simulink model "Y3Tiltrotor_sim3_INDI"  (R2025a)
settings: Solver=ode4  StartTime=0.0  StopTime=70  FixedStep=uavParam.sampleTime  RelTol=1e-3
PreLoadFcn:
  | filepath  = fileparts(get_param(bdroot, 'FileName'))
  | cd(filepath);
InitFcn:
  | Init_sim_INDI;
values from neighbouring files (symbols this model uses):
  control = struct    [Init_sim_INDI.m]
  env = struct    [InitData.m]
  flightState = struct    [Init_sim_INDI.m]
  FWSpeed0 = 15    [Init_sim_INDI.m]
  k_lpf_p = 50    [Init_sim_INDI.m]
  k_lpf_q = 80    [Init_sim_INDI.m]
  k_lpf_r = 5    [Init_sim_INDI.m]
  k_lpf_u = 10    [Init_sim_INDI.m]
  k_lpf_v = 1    [Init_sim_INDI.m]
  k_lpf_w = 50    [Init_sim_INDI.m]
  k_p = 5    [Init_sim_INDI.m]
  k_q = 20    [Init_sim_INDI.m]
  k_r = 1.5    [Init_sim_INDI.m]
  k_u = 0.5    [Init_sim_INDI.m]
  k_v = 0.5    [Init_sim_INDI.m]
  k_w = 2    [Init_sim_INDI.m]
  uavParam = struct    [InitData.m]
undefined symbols (not defined in the file or in its folder): ControlSampleTime, F, Light, MIL, Newton, Raphson
libraries: slpidlib x28, SignalEditorBlockLib x12, simulink x6, aerolibtransform2 x3, sharedtransform x3, robotcorelib x3, matrix_library x3, aerolibasang x2, aerolibutil x2, aerolibwind2 x2, shared6dof x1, aerolibatmos2 x1
(part 1 of 7)
settings Model: Creator=YuXinchen  LastModifiedBy=11696
settings SolverCC: AlgebraicLoopSolver=TrustRegion
settings DataIOCC: ReturnWorkspaceOutputs=off
settings DebuggingCC: UnconnectedInputMsg=warning  UnconnectedOutputMsg=warning  UnconnectedLineMsg=warning  UnderSpecifiedDimensionMsg=warning
settings ModelReferenceCC: EnableRefExpFcnMdlSchedulingChecks=on
settings RTWCC: GPUComputeCapability=3.5  DLArmComputeVersion=19.05

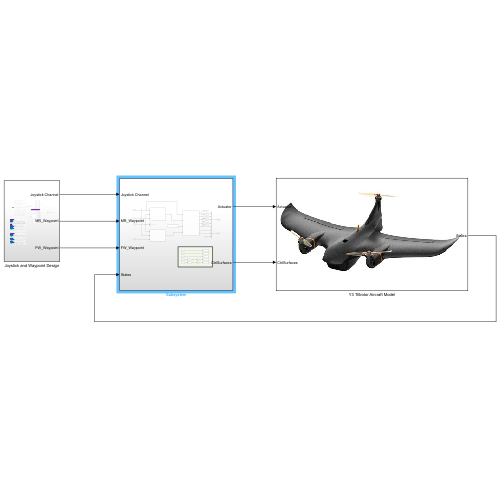
[thumbnail: Simulink's stored preview of the top-level diagram]
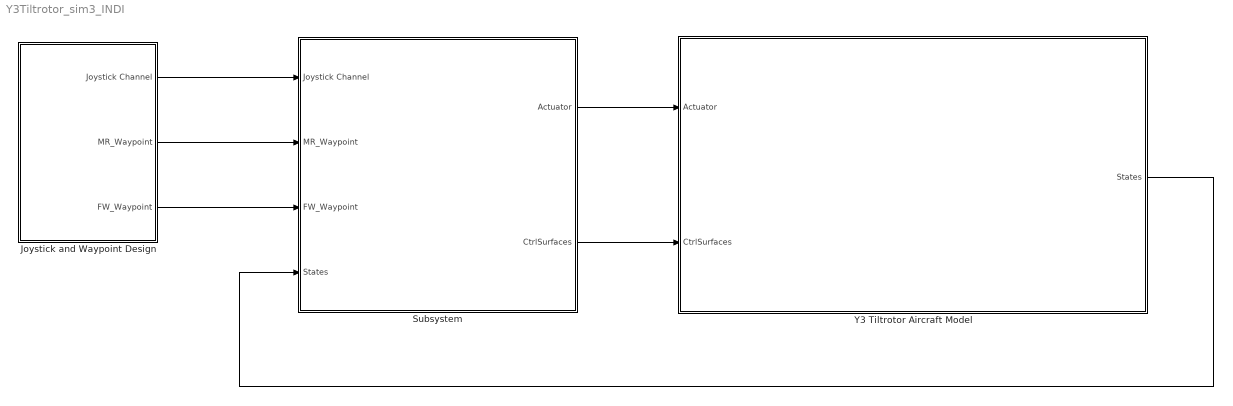
== system Y3Tiltrotor_sim3_INDI ==
  Joystick and Waypoint Design : Subsystem
  Subsystem : Subsystem
  Y3 Tiltrotor Aircraft Model : Subsystem
      mask Display: image('Y3Tiltrotor.jpg');
  wires:
  Subsystem/1(Actuator) -> Y3 Tiltrotor Aircraft Model/1(Actuator)
  Subsystem/2(CtrlSurfaces) -> Y3 Tiltrotor Aircraft Model/2(CtrlSurfaces)
  Y3 Tiltrotor Aircraft Model/1(States) -> Subsystem/4(States)
  Joystick and Waypoint Design/1(Joystick Channel) -> Subsystem/1(Joystick Channel)
  Joystick and Waypoint Design/2(MR_Waypoint) -> Subsystem/2(MR_Waypoint)
  Joystick and Waypoint Design/3(FW_Waypoint) -> Subsystem/3(FW_Waypoint)

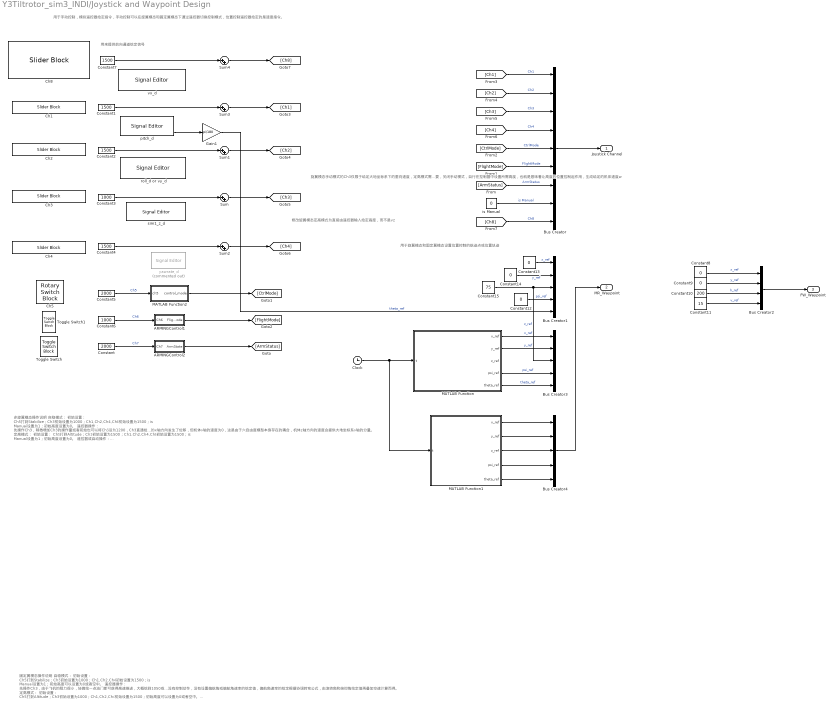
== system Y3Tiltrotor_sim3_INDI/Joystick and Waypoint Design ==
  note: 旋翼模态手动模式的Ch3仅限于给定大地坐标系下的垂向速度，定高模式需要，关闭手动模式，自行在控制器中设置所需高度，也就是意味着让高度的位置控制起作用，生成给定的机体速度w
  note: 用来提供前向通道给定信号
  note: 用于手动控制，模拟遥控器给定指令，手动控制可以在旋翼模态和固定翼模态下通过遥控器切换控制模式，位置控制遥控器给定的是速度指令。
  note: 用于旋翼模态和固定翼模态设置位置控制的航迹点或位置轨迹
  note: 固定翼模态操作说明
      |
      | 自稳模式：
      | 初始设置： Ch5打到Stabilize；Ch3初始设置为1000；Ch1,Ch2,Ch4初始设置为1500；is Manual设置为1；初始高度可以设置为0或者空中。
      | 遥控器操作： 先操作Ch3，由于飞机的阻力很小，轻微给一点油门即可获得高速推进，大概给到1050或1100即可；Ch1控制俯仰运动，在有油门的情况下进行操纵，增大Ch1即增大给定俯仰角，反之减小，抬头为正，低头为负；Ch2控制滚转运动，在有油门的情况下进行操纵，增大Ch2即增大给定滚转角，反之减小，向右滚转为正，向左滚转为负；Ch4没有控制动作，没有设置偏航角或偏航角速率的给定值，偏航角速率的给定根据协调转弯公式，由滚转角和俯仰角给定值再叠加空速计算而得。
      | 定高模式：
      | 初始设置： Ch5打到Altitude；Ch3初始设置为1000；Ch1,Ch2,Ch4初始设置为1500；初始高度可以设置为0或者空中。
      | 遥控器或自动操作： 此模式下无论是遥控器还是自动飞行，Ch3的操作和自稳模式一致；Ch2和Ch4的操作和自稳模式一致。当is Manual设置为1时（手动），Ch1控制飞机的垂向速度，增大Ch1即增大给定垂向速度，反之减小；当is Manual设置为0时（自动），Ch1不起作用，由FW_Waypoint给定飞机的飞行高度h_ref，高度控制器中的高度位置控制起作用。
      | 定速模式 ：
      | 初始设置： Ch5打到Position；Ch3初始设置可以为1000；Ch1,Ch2,Ch4初始设置为1500；初始高度可以设置为0或者空中。
      | 遥控器或自动操作： 此模式下无论是遥控器还是自动飞行，Ch2和Ch4的操作和自稳模式一致。当is Manual设置为1时（手动），Ch3控制飞机的空速，定速模式遥控器给定空速变化范围设置为15-25m/s；Ch1控制飞机的垂向速度，增大Ch1即增大给定垂向速度，反之减小。当is Manual设置为0时（自动），Ch1和Ch3都不起作用，对应于定速模式的给定变成了由FW_Waypoint给定飞机的飞行高度h_ref和飞行速度v_ref，在自动模式下，也可以调整CoupledControl的值来设置是否开启总能量控制。
  note: 多旋翼模态操作说明
      |
      | 自稳模式：
      | 初始设置： Ch5打到Stabilize；Ch3初始设置为1000；Ch1,Ch2,Ch4,Ch8初始设置为1500；is Manual设置为1；初始高度设置为0。
      | 遥控器操作： 先操作Ch3，稍微增加Ch3的操作量或者初始也可以将Ch3设为1200，Ch3直通给到油门量，飞行器将获得持续的推力，当达到想要的高度后可以适当降低油门量使其能大致平衡重力，也可以保持垂向飞行的状态操作其他通道。Ch1控制俯仰通道，给定俯仰角；Ch2控制滚转通道，给定滚转角；Ch4控制偏航通道，给定偏航角速率，Ch8控制前向通道，给定机体坐标系前向速度。由于所设计的控制逻辑是通过前两个旋翼的油门和倾转角来控制前向通道，与俯仰通道解耦，所以在自稳模式的前向通道控制过程中，俯仰角可以始终为0，可以自行设定；在俯仰通道的控制过程中，前向速度也可以设定为0，但通常会发现无人机的x轴方向发生了位移，但机体x轴的速度为0，这是由于六自由度模型本身存在的耦合，机体z轴方向的速度会提供大地坐标系x轴的分量。
      | 定高模式：
      | 初始设置： Ch5打到Altitude；Ch3初始设置为1500；Ch1,Ch2,Ch4,Ch8初始设置为1500；is Manual设置为1；初始高度设置为0。
      | 遥控器或自动操作： 此模式下只有Ch3和自稳模式不一样，其他通道基本保持一致。Ch3控制垂向速度，给定为大地坐标系下z轴的速度。其他通道做动作时，通常将Ch3置为1500，即将无人机保持定高飞行，高度不变的情况下做其他动作。
      | 定点模式 ：
      | 初始设置： Ch5打到Position；Ch3初始设置可以为1500；Ch1,Ch2,Ch4 ,Ch8 初始设置为1500；初始高度可以设置为0。
      | 遥控器或自动操作： 此模式下无论是遥控器还是自动飞行，Ch1和Ch4,Ch8的操作和自稳模式一致。当is Manual设置为1时（手动），Ch3控制垂向速度，和定高模式保持一致；Ch2控制横侧向通道，给定为飞机机体坐标系y轴的速度（横向速度）。当is Manual设置为0时（自动），Ch1, Ch2, Ch3 ,Ch4 ,Ch8都不起作用，对应于定速模式的给定变成了由FW_Waypoint给定飞机的x_ref,y_ref,z_ref,psi_ref的给定。
  note: 修改旋翼模态定高模式为直接由遥控器输入给定高度，而不是vz
  ARMINGControl1 : Subsystem
  ARMINGControl2 : Subsystem
  Bus Creator : BusCreator  Inputs=9
  Bus Creator1 : BusCreator  Inputs=5
  Bus Creator2 : BusCreator  Inputs=4
  Bus Creator3 : BusCreator  Inputs=5
  Bus Creator4 : BusCreator  Inputs=5
  Ch{1..4,8} (5 alike) : SliderBlock  ScaleMin=1000  ScaleMax=2000  TickInterval=200
  Ch5 : RotarySwitchBlock
  Clock : Clock
  Constant : Constant  Value=2000
  Constant{1..2,4,7} (4 alike) : Constant  Value=1500
  Constant10 : Constant  Value=200
  Constant11 : Constant  Value=15
  Constant{8..9,12..14} (5 alike) : Constant  Value=0
  Constant15 : Constant  Value=75
  Constant3 : Constant  Value=1000
  Constant5 : Constant  Value=2000
  Constant6 : Constant  Value=1000
  Gain1 : Gain  Gain=pi/180
  MATLAB Function : MATLAB Function  TreatAsAtomicUnit=on
  MATLAB Function1 : MATLAB Function  TreatAsAtomicUnit=on
  MATLAB Function2 : MATLAB Function  TreatAsAtomicUnit=on
  Sum{,1..4} (5 alike) : Sum  Inputs=|++
  Toggle Switch : ToggleSwitchBlock
  Toggle Switch1 : ToggleSwitchBlock
  is Manual : Constant  Value=0
  pitch_d : SignalEditorBlockLib/Signal Editor  FileName=pitch_d.mat  ActiveScenario=Test  ActiveSignal=俯仰角测试-遥控器  IsBus=off  OutputBusObjectStr=Bus: BusObject  SampleTime=0  ZeroCross=off  OutputAfterFinalValue=Setting to zero  Unit=inherit  PreserveSignalName=on  ApplySigPropsToAllScenarios=on  ApplySigPropsToAllSignals=on  SignalPropertySource=Dialog parameters
  roll_d or vy_d : SignalEditorBlockLib/Signal Editor  FileName=roll_d.mat  ActiveScenario=Test  ActiveSignal=定高-滚转角测试-遥控器  IsBus=off  OutputBusObjectStr=Bus: BusObject  SampleTime=0  ZeroCross=off  OutputAfterFinalValue=Setting to zero  Unit=inherit  PreserveSignalName=on  ApplySigPropsToAllScenarios=on  ApplySigPropsToAllSignals=on  SignalPropertySource=Dialog parameters
  sim1_z_d : SignalEditorBlockLib/Signal Editor  FileName=vz_d.mat  ActiveScenario=Test  ActiveSignal=直接给定高度-遥控器  IsBus=off  OutputBusObjectStr=Bus: BusObject  SampleTime=0  ZeroCross=off  OutputAfterFinalValue=Setting to zero  Unit=inherit  PreserveSignalName=on  ApplySigPropsToAllScenarios=on  ApplySigPropsToAllSignals=on  SignalPropertySource=Dialog parameters
  vx_d : SignalEditorBlockLib/Signal Editor  FileName=vx_d.mat  ActiveScenario=Test  ActiveSignal=定点-前向速度测试-遥控器  IsBus=off  OutputBusObjectStr=Bus: BusObject  SampleTime=0  ZeroCross=off  OutputAfterFinalValue=Setting to zero  Unit=inherit  PreserveSignalName=on  ApplySigPropsToAllScenarios=on  ApplySigPropsToAllSignals=off  SignalPropertySource=Dialog parameters
  yawrate_d : SignalEditorBlockLib/Signal Editor  Commented=on  FileName=untitled.mat  ActiveScenario=Scenario  ActiveSignal=Signal 1  IsBus=off  OutputBusObjectStr=Bus: BusObject  SampleTime=0  ZeroCross=off  OutputAfterFinalValue=Setting to zero  Unit=inherit  PreserveSignalName=on  ApplySigPropsToAllScenarios=on  ApplySigPropsToAllSignals=off  SignalPropertySource=Dialog parameters
  Joystick Channel : Outport
  MR_Waypoint : Outport  Port=2
  FW_Waypoint : Outport  Port=3
  wires:
  Constant5/1 -> MATLAB Function2/1(ch5)  "Ch5"
  Constant/1 -> ARMINGControl2/1(Ch7)  "Ch7"
  Constant6/1 -> ARMINGControl1/1(Ch6)  "Ch6"
  ARMINGControl2/1(ArmState) -> [ArmStatus]
  MATLAB Function2/1(control_mode) -> [CtrlMode]
  ARMINGControl1/1(FlightMode) -> [FlightMode]
  Bus Creator/1 -> Joystick Channel/1
  [CtrlMode] -> Bus Creator/5  "CtrlMode"
  [FlightMode] -> Bus Creator/6  "FlightMode"
  [ArmStatus] -> Bus Creator/7  "ArmStatus"
  [Ch1] -> Bus Creator/1  "Ch1"
  [Ch2] -> Bus Creator/2  "Ch2"
  [Ch3] -> Bus Creator/3  "Ch3"
  [Ch4] -> Bus Creator/4  "Ch4"
  is Manual/1 -> Bus Creator/8  "is Manual"
  Constant3/1 -> Sum/1
  Constant2/1 -> Sum1/1
  Constant4/1 -> Sum2/1
  Sum1/1 -> [Ch2]
  Sum/1 -> [Ch3]
  Sum2/1 -> [Ch4]
  Sum3/1 -> [Ch1]
  Constant1/1 -> Sum3/1
  [Ch8] -> Bus Creator/9  "Ch8"
  Sum4/1 -> [Ch8]
  Constant7/1 -> Sum4/1
  Constant14/1 -> Bus Creator1/2  "y_ref"
  Constant13/1 -> Bus Creator1/1  "x_ref"
  Clock/1 -> MATLAB Function1/1(t), MATLAB Function/1(t)
  Constant12/1 -> Bus Creator1/4  "psi_ref"
  Constant11/1 -> Bus Creator2/4  "v_ref"
  Constant8/1 -> Bus Creator2/1  "x_ref"
  Constant10/1 -> Bus Creator2/3  "h_ref"
  Bus Creator2/1 -> FW_Waypoint/1
  Constant9/1 -> Bus Creator2/2  "y_ref"
  Constant15/1 -> Bus Creator1/3, Bus Creator3/3  "z_ref"
  pitch_d/3 -> Gain1/1
  Gain1/1 -> Bus Creator1/5  "theta_ref"
  MATLAB Function/1(x_ref) -> Bus Creator3/1  "x_ref"
  MATLAB Function/2(y_ref) -> Bus Creator3/2  "y_ref"
  MATLAB Function/4(psi_ref) -> Bus Creator3/4  "psi_ref"
  MATLAB Function/5(theta_ref) -> Bus Creator3/5  "theta_ref"
  MATLAB Function1/3(z_ref) -> Bus Creator4/3
  MATLAB Function1/1(x_ref) -> Bus Creator4/1
  MATLAB Function1/2(y_ref) -> Bus Creator4/2
  MATLAB Function1/4(psi_ref) -> Bus Creator4/4
  MATLAB Function1/5(theta_ref) -> Bus Creator4/5
  Bus Creator4/1 -> MR_Waypoint/1

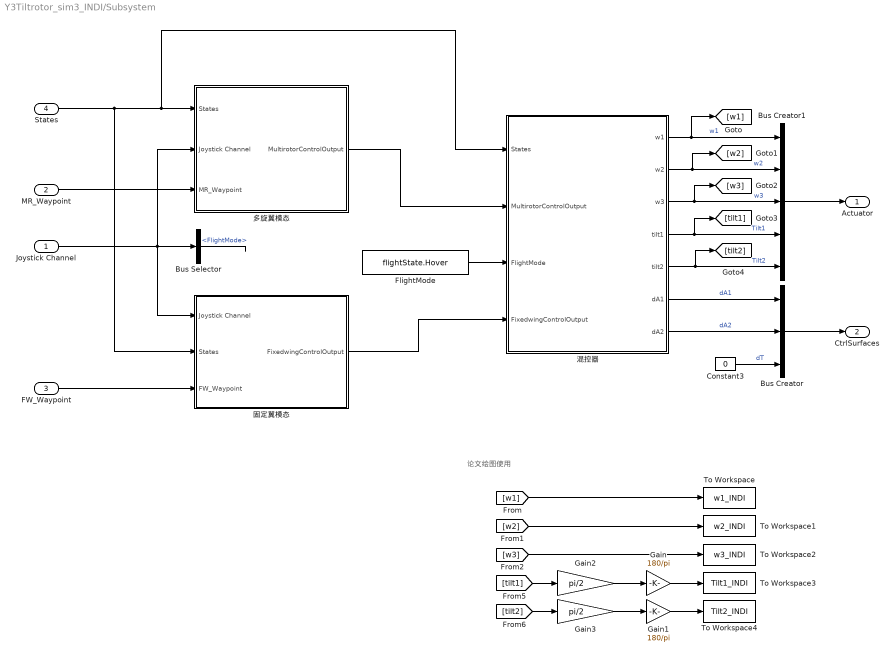
== system Y3Tiltrotor_sim3_INDI/Subsystem ==
  note: 论文绘图使用
  Joystick Channel : Inport
  MR_Waypoint : Inport  Port=2
  FW_Waypoint : Inport  Port=3
  States : Inport  Port=4
  Bus Creator : BusCreator  Inputs=3
  Bus Creator1 : BusCreator  Inputs=5
  Bus Selector : BusSelector  OutputSignals=FlightMode
  Constant3 : Constant  Value=0
  FlightMode : Constant  Value=flightState.Hover
  Gain : Gain  Gain=180/pi
  Gain1 : Gain  Gain=180/pi
  Gain2 : Gain  Gain=pi/2
  Gain3 : Gain  Gain=pi/2
  To Workspace : ToWorkspace  VariableName=w1_INDI  SampleTime=-1
      settings: Save2DSignal=2-D array (concatenate along first dimension)
  To Workspace1 : ToWorkspace  VariableName=w2_INDI  SampleTime=-1
      settings: Save2DSignal=2-D array (concatenate along first dimension)
  To Workspace2 : ToWorkspace  VariableName=w3_INDI  SampleTime=-1
      settings: Save2DSignal=2-D array (concatenate along first dimension)
  To Workspace3 : ToWorkspace  VariableName=Tilt1_INDI  SampleTime=-1
      settings: Save2DSignal=2-D array (concatenate along first dimension)
  To Workspace4 : ToWorkspace  VariableName=Tilt2_INDI  SampleTime=-1
      settings: Save2DSignal=2-D array (concatenate along first dimension)
  固定翼模态 : Subsystem
  多旋翼模态 : Subsystem
  混控器 : Subsystem
  Actuator : Outport
  CtrlSurfaces : Outport  Port=2
  wires:
  Constant3/1 -> Bus Creator/3  "dT"
  混控器/5(tilt2) -> [tilt2], Bus Creator1/5  "Tilt2"
  混控器/4(tilt1) -> [tilt1], Bus Creator1/4  "Tilt1"
  Bus Creator/1 -> CtrlSurfaces/1
  Bus Creator1/1 -> Actuator/1
  States/1 -> 混控器/1(States), 多旋翼模态/1(States), 固定翼模态/2(States)
  混控器/1(w1) -> [w1], Bus Creator1/1  "w1"
  混控器/2(w2) -> [w2], Bus Creator1/2  "w2"
  混控器/3(w3) -> [w3], Bus Creator1/3  "w3"
  混控器/7(dA2) -> Bus Creator/2  "dA2"
  混控器/6(dA1) -> Bus Creator/1  "dA1"
  FlightMode/1 -> 混控器/3(FlightMode)
  Joystick Channel/1 -> Bus Selector/1, 多旋翼模态/2(Joystick Channel), 固定翼模态/1(Joystick Channel)
  Bus Selector/1 -> ?  "<FlightMode>"
  MR_Waypoint/1 -> 多旋翼模态/3(MR_Waypoint)
  FW_Waypoint/1 -> 固定翼模态/3(FW_Waypoint)
  多旋翼模态/1(MultirotorControlOutput) -> 混控器/2("MultirotorControlOutput ")
  固定翼模态/1(FixedwingControlOutput) -> 混控器/4("FixedwingControlOutput ")
  Gain3/1 -> Gain1/1
  Gain2/1 -> Gain/1
  Gain1/1 -> To Workspace4/1
  [w1] -> To Workspace/1
  [w2] -> To Workspace1/1
  [w3] -> To Workspace2/1
  Gain/1 -> To Workspace3/1
  [tilt2] -> Gain3/1
  [tilt1] -> Gain2/1

== system Y3Tiltrotor_sim3_INDI/Y3 Tiltrotor Aircraft Model ==
  Actuator : Inport
  CtrlSurfaces : Inport  Port=2
  6DOF (Euler Angles) : shared6dof/6DOF (Euler Angles)  units=Metric (MKS)  mtype=Fixed  rep=Euler Angles  xme_0=ModelInit_PosE  Vm_0=ModelInit_VelB  eul_0=ModelInit_AngEuler  pm_0=ModelInit_RateB  mass_0=uavParam.geom.mass  mass_e=0.5  mass_f=2.0  inertia=eye(3).*[uavParam.inertia.Ixx; uavParam.inertia.Iyy; uavParam.inertia.Izz]  inertia_e=eye(3)  inertia_f=2*eye(3)  k_quat=1.0  vre_flag=on  abi_flag=off  aMode=aMode  xme_statename=''  Vm_statename=''  eul_statename=''  quat_statename=''  pm_statename=''  mass_statename=''
  Rate Transition : RateTransition
  Rate Transition1 : RateTransition
  States Bus : Subsystem
  Subsystem : Subsystem
  States : Outport
  wires:
  6DOF (Euler Angles)/1 -> States Bus/1(Ve)  "Ve"
  States Bus/1(States) -> Subsystem/3(States), States/1
  6DOF (Euler Angles)/8 -> States Bus/8(Abb)  "Abb"
  6DOF (Euler Angles)/7 -> States Bus/7(dw/dt)  "dw/dt"
  6DOF (Euler Angles)/6 -> States Bus/6(pqr)  "pqr"
  6DOF (Euler Angles)/5 -> States Bus/5(Vb)  "Vb"
  6DOF (Euler Angles)/4 -> States Bus/4(DCMbe)  "DCM"
  6DOF (Euler Angles)/3 -> States Bus/3(Euler)  "Euler"
  6DOF (Euler Angles)/2 -> States Bus/2(Xe)  "Xe"
  CtrlSurfaces/1 -> Rate Transition1/1
  Actuator/1 -> Rate Transition/1
  Subsystem/1(Fb) -> 6DOF (Euler Angles)/1  "F_b"
  Subsystem/2(Mb) -> 6DOF (Euler Angles)/2  "M_b"
  Subsystem/3(RotorParams) -> States Bus/9(RotorParams)
  Subsystem/4(Airspeed) -> States Bus/10(Airspeed)
  Rate Transition1/1 -> Subsystem/2(CtrlSurfaces)
  Rate Transition/1 -> Subsystem/1(Actuator)

== system Y3Tiltrotor_sim3_INDI/Joystick and Waypoint Design/ARMINGControl1 ==
  Ch6 : Inport
  Compare To Constant3 : simulink/Logic and Bit Operations/Compare To Constant  relop=>=  const=uint16(1400)  OutDataTypeStr=boolean
  FlightMode : Outport  VectorParamsAs1DForOutWhenUnconnected=off
  wires:
  Ch6/1 -> Compare To Constant3/1
  Compare To Constant3/1 -> FlightMode/1

== system Y3Tiltrotor_sim3_INDI/Joystick and Waypoint Design/ARMINGControl2 ==
  Ch7 : Inport
  Compare To Constant3 : simulink/Logic and Bit Operations/Compare To Constant  relop=>=  const=uint16(1400)  OutDataTypeStr=boolean
  ArmState : Outport  VectorParamsAs1DForOutWhenUnconnected=off
  wires:
  Compare To Constant3/1 -> ArmState/1
  Ch7/1 -> Compare To Constant3/1

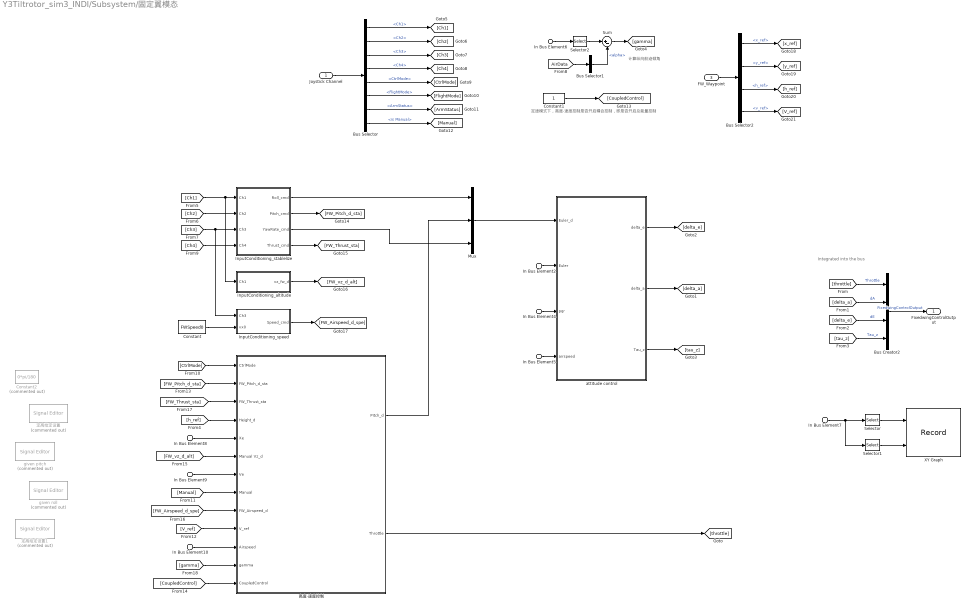
== system Y3Tiltrotor_sim3_INDI/Subsystem/固定翼模态 ==
  note: 计算纵向航迹倾角
  note: Integrated into the bus
  note: 定速模式下，高度-速度控制是否开启耦合控制，即是否开启总能量控制
  Joystick Channel : Inport
  In Bus Element5 : Inport  Port=2  PortName=States  Element=Airspeed
  In Bus Element10 : Inport  Port=2  PortName=States  Element=Airspeed
  In Bus Element7 : Inport  Port=2  PortName=States  Element=Xe
  In Bus Element8 : Inport  Port=2  PortName=States  Element=Xe
  In Bus Element2 : Inport  Port=2  PortName=States  Element=Euler
  In Bus Element6 : Inport  Port=2  PortName=States  Element=Euler
  In Bus Element9 : Inport  Port=2  PortName=States  Element=Ve
  In Bus Element4 : Inport  Port=2  PortName=States  Element=pqr
  FW_Waypoint : Inport  Port=3
  Bus Creator2 : BusCreator  Inputs=4
  Bus Selector : BusSelector  OutputSignals=Ch1,Ch2,Ch3,Ch4,CtrlMode,FlightMode,ArmStatus,is Manual
  Bus Selector1 : BusSelector  OutputSignals=alpha
  Bus Selector2 : BusSelector  OutputSignals=x_ref,y_ref,h_ref,v_ref
  Constant : Constant  Value=FWSpeed0
  Constant1 : Constant
  Constant2 : Constant  Commented=on  Value=0*pi/180
  InputConditioning_altitude : Subsystem
  InputConditioning_speed : Subsystem
  InputConditioning_stablelize : Subsystem
  Mux : Mux  Inputs=3
  Selector : Selector  InputPortWidth=3  IndexOptions=Index vector (dialog)  Indices=1  OutputSizes=1
  Selector1 : Selector  InputPortWidth=3  IndexOptions=Index vector (dialog)  Indices=2  OutputSizes=1
  Selector2 : Selector  InputPortWidth=3  IndexOptions=Index vector (dialog)  Indices=2  OutputSizes=1
  Sum : Sum  Inputs=|+-
  XY Graph : Record  NumPorts=2.0  FileSettingsInternal="{\"entries\":[{\"content\":{\"excelSettings\":{\"content\":{},\"type\":\"Streamout.ExcelSettings\"},\"parquetSettings\":{\"content\":{},\"type\":\"Streamout.ParquetSettings\"}},\"type\":\"Streamout.FileSettingStorage\",\"uuid\":\"\"}],\"packageUris\":[\"http:\\/\\/schema.mathworks.com\\/mf0\\/streamout_blocks\\/R2020a\"],\"version\":\"1.0\"}"  FrameSettings=[0, 0]  Layout=OverlayBottom  SignalsInternal="{\"entries\":[{\"content\":{\"signals\":[{\"content\":{\"blockPath\":[],\"dimensions\":[1],\"domain\":\"\",\"lineColor\":\"#edb120\",\"lineWidth\":2,\"port\":1,\"sid\":[\"\"],\"signalID\":1,\"signalName\":\"Selector\"},\"type\":\"RecordBlkView.Signal\",\"uuid\":\"\"},{\"content\":{\"blockPath\":[],\"dimensions\":[1],\"domain\":\"\",\"lineColor\":\"#7e2f8e\",\"lineWidth\":2,\"port\":2,\"sid\":[\"\"],\"signalID\":2,\"signalName\":\"Selector1\"},\"type\":\"RecordBlkView.Signal\",\"uuid\":\"\"}]},\"type\":\"RecordBlkView.InputSignals\",\"uuid\":\"\"}],\"packageUris\":[\"http:\\/\\/schema.mathworks.com\\/mf0\\/streamout_blocks\\/R2020a\"],\"version\":\"1.0\"}"  VisualizationBindings="{\"xyplotplugin\":{\"info\":[{\"series\":[],\"subplotID\":1}]}}"  CompatibilityTag=XY
  attitude control : Subsystem
  given pitch : SignalEditorBlockLib/Signal Editor  Commented=on  FileName=given pitch.mat  ActiveScenario=Scenario  ActiveSignal=Signal 1  IsBus=off  OutputBusObjectStr=Bus: BusObject  SampleTime=0  Interpolate=off  ZeroCross=off  OutputAfterFinalValue=Setting to zero  Unit=inherit  PreserveSignalName=on  ApplySigPropsToAllScenarios=on  ApplySigPropsToAllSignals=off  SignalPropertySource=Dialog parameters
  given roll : SignalEditorBlockLib/Signal Editor  Commented=on  FileName=given roll.mat  ActiveScenario=Scenario  ActiveSignal=Signal 1  IsBus=off  OutputBusObjectStr=Bus: BusObject  SampleTime=-1  ZeroCross=off  OutputAfterFinalValue=Setting to zero  Unit=inherit  PreserveSignalName=on  ApplySigPropsToAllScenarios=on  ApplySigPropsToAllSignals=off  SignalPropertySource=Dialog parameters
  定高给定设置 : SignalEditorBlockLib/Signal Editor  Commented=on  FileName=E:\1-实验室相关\1-科研\10-倾转旋翼无人机\SmallTiltrotorUAV\v2.0\given Fixed Height.mat  ActiveScenario=Scenario  ActiveSignal=Signal 1  IsBus=off  OutputBusObjectStr=Bus: BusObject  SampleTime=0  ZeroCross=off  OutputAfterFinalValue=Setting to zero  Unit=inherit  PreserveSignalName=on  ApplySigPropsToAllScenarios=on  ApplySigPropsToAllSignals=off  SignalPropertySource=Dialog parameters
  定高给定设置1 : SignalEditorBlockLib/Signal Editor  Commented=on  FileName=E:\1-实验室相关\1-科研\10-倾转旋翼无人机\SmallTiltrotorUAV\v2.0\given Fixed Height.mat  ActiveScenario=Scenario  ActiveSignal=Signal 1  IsBus=off  OutputBusObjectStr=Bus: BusObject  SampleTime=0  ZeroCross=off  OutputAfterFinalValue=Setting to zero  Unit=inherit  PreserveSignalName=on  ApplySigPropsToAllScenarios=on  ApplySigPropsToAllSignals=off  SignalPropertySource=Dialog parameters
  高度-速度控制 : Subsystem
  FixedwingControlOutput : Outport
  wires:
  Mux/1 -> attitude control/1(Euler_d)
  In Bus Element2/1 -> attitude control/2(Euler)
  In Bus Element4/1 -> attitude control/3(pqr)
  attitude control/1(delta_e) -> [delta_e]
  InputConditioning_stablelize/3(YawRate_cmd) -> Mux/3
  attitude control/2(delta_a) -> [delta_a]
  attitude control/3(Tau_z) -> [tau_z]
  In Bus Element5/1 -> attitude control/4(airspeed)
  [tau_z] -> Bus Creator2/4  "Tau_z"
  [delta_e] -> Bus Creator2/3  "dE"
  [throttle] -> Bus Creator2/1  "Throttle"
  [delta_a] -> Bus Creator2/2  "dA"
  Bus Creator2/1 -> FixedwingControlOutput/1  "FixedwingControlOutput"
  Joystick Channel/1 -> Bus Selector/1
  In Bus Element6/1 -> Selector2/1
  Selector2/1 -> Sum/1
  Sum/1 -> [gamma]
  [AirData] -> Bus Selector1/1
  Bus Selector1/1 -> Sum/2  "<alpha>"
  Selector/1 -> XY Graph/1
  Selector1/1 -> XY Graph/2
  In Bus Element7/1 -> Selector1/1, Selector/1
  Bus Selector/8 -> [Manual]  "<is Manual>"
  Bus Selector/7 -> [ArmStatus]  "<ArmStatus>"
  Bus Selector/6 -> [FlightMode]  "<FlightMode>"
  Bus Selector/5 -> [CtrlMode]  "<CtrlMode>"
  Bus Selector/4 -> [Ch4]  "<Ch4>"
  Bus Selector/3 -> [Ch3]  "<Ch3>"
  Bus Selector/1 -> [Ch1]  "<Ch1>"
  Bus Selector/2 -> [Ch2]  "<Ch2>"
  Constant1/1 -> [CoupledControl]
  [Ch1] -> InputConditioning_altitude/1(Ch1), InputConditioning_stablelize/1(Ch1)
  [Ch2] -> InputConditioning_stablelize/2(Ch2)
  [Ch3] -> InputConditioning_speed/1(Ch3), InputConditioning_stablelize/3(Ch3)
  [Ch4] -> InputConditioning_stablelize/4(Ch4)
  InputConditioning_stablelize/4(Thrust_cmd) -> [FW_Thrust_sta]
  InputConditioning_stablelize/2(Pitch_cmd) -> [FW_Pitch_d_sta]
  InputConditioning_altitude/1(vz_fw_d) -> [FW_vz_d_alt]
  Constant/1 -> InputConditioning_speed/2(vx0)
  InputConditioning_speed/1(Speed_cmd) -> [FW_Airspeed_d_spe]
  [CtrlMode] -> 高度-速度控制/1(CtrlMode)
  [FW_Pitch_d_sta] -> 高度-速度控制/2(FW_Pitch_d_sta)
  [FW_Thrust_sta] -> 高度-速度控制/3(FW_Thrust_sta)
  In Bus Element8/1 -> 高度-速度控制/5(Xe)
  In Bus Element9/1 -> 高度-速度控制/7(Ve)
  [FW_vz_d_alt] -> 高度-速度控制/6(Manual Vz_d)
  [Manual] -> 高度-速度控制/8(Manual)
  [FW_Airspeed_d_spe] -> 高度-速度控制/9(FW_Airspeed_d)
  In Bus Element10/1 -> 高度-速度控制/11(Airspeed)
  [gamma] -> 高度-速度控制/12(gamma)
  [CoupledControl] -> 高度-速度控制/13(CoupledControl)
  高度-速度控制/1(Pitch_d) -> Mux/2
  高度-速度控制/2(Throttle) -> [throttle]
  InputConditioning_stablelize/1(Roll_cmd) -> Mux/1
  [h_ref] -> 高度-速度控制/4(Height_d)
  FW_Waypoint/1 -> Bus Selector2/1
  Bus Selector2/1 -> [x_ref]  "<x_ref>"
  Bus Selector2/2 -> [y_ref]  "<y_ref>"
  Bus Selector2/3 -> [h_ref]  "<h_ref>"
  Bus Selector2/4 -> [V_ref]  "<v_ref>"
  [V_ref] -> 高度-速度控制/10(V_ref)

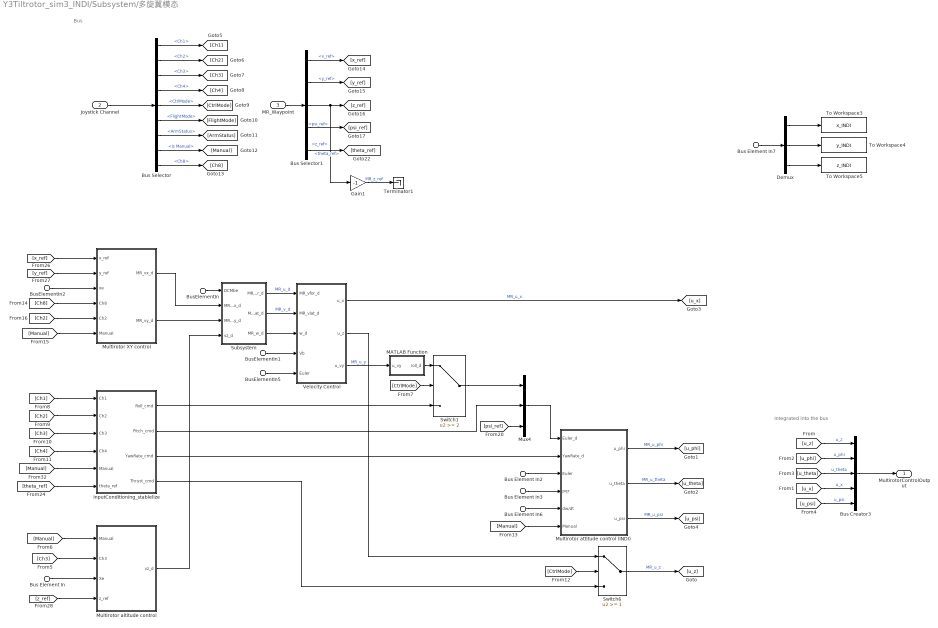
== system Y3Tiltrotor_sim3_INDI/Subsystem/多旋翼模态 ==
  note: Bus
  note: Integrated into the bus
  Bus Element In : Inport  PortName=States  Element=Xe
  Bus Element In7 : Inport  PortName=States  Element=Xe
  BusElementIn2 : Inport  PortName=States  Element=Xe
  Bus Element In2 : Inport  PortName=States  Element=Euler
  BusElementIn5 : Inport  PortName=States  Element=Euler
  Bus Element In3 : Inport  PortName=States  Element=pqr
  BusElementIn : Inport  PortName=States  Element=DCMbe
  BusElementIn1 : Inport  PortName=States  Element=Vb
  Bus Element In6 : Inport  PortName=States  Element=dw/dt
  Joystick Channel : Inport  Port=2
  MR_Waypoint : Inport  Port=3
  Bus Creator3 : BusCreator  Inputs=5
  Bus Selector : BusSelector  OutputSignals=Ch1,Ch2,Ch3,Ch4,CtrlMode,FlightMode,ArmStatus,is Manual,Ch8
  Bus Selector1 : BusSelector  OutputSignals=x_ref,y_ref,z_ref,psi_ref,theta_ref
  Demux : Demux  Outputs=3
  Gain1 : Gain  Gain=-1
  InputConditioning_stablelize : Subsystem
  MATLAB Function : MATLAB Function  TreatAsAtomicUnit=on
  Multirotor XY control : Subsystem
  Multirotor altitude control : Subsystem
  Multirotor attitude control (INDI) : Subsystem
  Mux4 : Mux  Inputs=3
  Subsystem : Subsystem
  Switch1 : Switch  Threshold=2  SaturateOnIntegerOverflow=off  InputSameDT=off
  Switch6 : Switch  Threshold=1  SaturateOnIntegerOverflow=off  InputSameDT=off
  Terminator1 : Terminator
  To Workspace3 : ToWorkspace  VariableName=x_INDI  SampleTime=-1
      settings: Save2DSignal=2-D array (concatenate along first dimension)
  To Workspace4 : ToWorkspace  VariableName=y_INDI  SampleTime=-1
      settings: Save2DSignal=2-D array (concatenate along first dimension)
  To Workspace5 : ToWorkspace  VariableName=z_INDI  SampleTime=-1
      settings: Save2DSignal=2-D array (concatenate along first dimension)
  Velocity Control : Subsystem
  MultirotorControlOutput : Outport
  wires:
  Bus Element In/1 -> Multirotor altitude control/3(Xe)
  Bus Element In2/1 -> Multirotor attitude control (INDI)/3(Euler)
  Bus Element In3/1 -> Multirotor attitude control (INDI)/4(pqr)
  Multirotor attitude control (INDI)/1(u_phi) -> [u_phi]  "MR_u_phi"
  Multirotor attitude control (INDI)/2(u_theta) -> [u_theta]  "MR_u_theta"
  Multirotor attitude control (INDI)/3(u_psi) -> [u_psi]  "MR_u_psi"
  [u_phi] -> Bus Creator3/2  "u_phi"
  [u_z] -> Bus Creator3/1  "u_z"
  [u_x] -> Bus Creator3/4  "u_x"
  [u_theta] -> Bus Creator3/3  "u_theta"
  [u_psi] -> Bus Creator3/5  "u_psi"
  Bus Creator3/1 -> MultirotorControlOutput/1
  Joystick Channel/1 -> Bus Selector/1
  Bus Selector/1 -> [Ch1]  "<Ch1>"
  Bus Selector/2 -> [Ch2]  "<Ch2>"
  Bus Selector/3 -> [Ch3]  "<Ch3>"
  Bus Selector/4 -> [Ch4]  "<Ch4>"
  Bus Selector/5 -> [CtrlMode]  "<CtrlMode>"
  Bus Selector/6 -> [FlightMode]  "<FlightMode>"
  Bus Selector/7 -> [ArmStatus]  "<ArmStatus>"
  [Ch3] -> Multirotor altitude control/2(Ch3)
  Bus Selector/8 -> [Manual]  "<is Manual>"
  [Manual] -> Multirotor altitude control/1(Manual)
  Switch6/1 -> [u_z]  "MR_u_z"
  [Ch3] -> InputConditioning_stablelize/3(Ch3)
  [Ch4] -> InputConditioning_stablelize/4(Ch4)
  [CtrlMode] -> Switch1/2
  [CtrlMode] -> Switch6/2
  InputConditioning_stablelize/4(Thrust_cmd) -> Switch6/3
  InputConditioning_stablelize/3(YawRate_cmd) -> Multirotor attitude control (INDI)/2(YawRate_d)
  [Manual] -> Multirotor attitude control (INDI)/6(Manual)
  [Ch1] -> InputConditioning_stablelize/1(Ch1)
  [Ch2] -> InputConditioning_stablelize/2(Ch2)
  Bus Selector/9 -> [Ch8]  "<Ch8>"
  Mux4/1 -> Multirotor attitude control (INDI)/1(Euler_d)
  InputConditioning_stablelize/2(Pitch_cmd) -> Mux4/2
  InputConditioning_stablelize/1(Roll_cmd) -> Switch1/3
  MR_Waypoint/1 -> Bus Selector1/1
  Bus Selector1/1 -> [x_ref]  "<x_ref>"
  Bus Selector1/2 -> [y_ref]  "<y_ref>"
  Bus Selector1/3 -> Gain1/1, [z_ref]  "<z_ref>"
  Bus Selector1/4 -> [psi_ref]  "<psi_ref>"
  Bus Element In7/1 -> Demux/1
  Demux/1 -> To Workspace3/1
  Demux/2 -> To Workspace4/1
  Demux/3 -> To Workspace5/1
  BusElementIn/1 -> Subsystem/1(DCMbe)
  Multirotor altitude control/1(vz_d) -> Subsystem/4(vz_d)
  BusElementIn1/1 -> Velocity Control/4(Vb)
  Velocity Control/1(u_x) -> [u_x]  "MR_u_x"
  Velocity Control/2(u_z) -> Switch6/1
  [z_ref] -> Multirotor altitude control/4(z_ref)
  [psi_ref] -> Mux4/3
  Bus Selector1/5 -> [theta_ref]  "<theta_ref>"
  [Manual] -> InputConditioning_stablelize/5(Manual)
  [theta_ref] -> InputConditioning_stablelize/6(theta_ref)
  MATLAB Function/1(roll_d) -> Switch1/1
  Switch1/1 -> Mux4/1
  Velocity Control/3(u_vy) -> MATLAB Function/1(u_vy)  "MR_u_y"
  BusElementIn5/1 -> Velocity Control/5(Euler)
  Gain1/1 -> Terminator1/1  "MR_z_ref"
  Subsystem/1(MR_vfor_d) -> Velocity Control/1(MR_vfor_d)  "MR_u_d"
  Subsystem/2(MR_vlat_d) -> Velocity Control/2(MR_vlat_d)  "MR_v_d"
  Subsystem/3(MR_w_d) -> Velocity Control/3(w_d)
  Multirotor XY control/1(MR_vx_d) -> Subsystem/2(MR_vx_d)
  Multirotor XY control/2(MR_vy_d) -> Subsystem/3(MR_vy_d)
  Bus Element In6/1 -> Multirotor attitude control (INDI)/5(dw/dt)
  [Manual] -> Multirotor XY control/6(Manual)
  [Ch2] -> Multirotor XY control/5(Ch2)
  [Ch8] -> Multirotor XY control/4(Ch8)
  BusElementIn2/1 -> Multirotor XY control/3(xe)
  [y_ref] -> Multirotor XY control/2(y_ref)
  [x_ref] -> Multirotor XY control/1(x_ref)

== system Y3Tiltrotor_sim3_INDI/Subsystem/混控器 ==
  States : Inport
  "MultirotorControlOutput " : Inport  Port=2
  FlightMode : Inport  Port=3
  "FixedwingControlOutput " : Inport  Port=4
  Bus Selector : BusSelector  OutputSignals=dA1,dA2
  Bus Selector1 : BusSelector  OutputSignals=w1,w2,w3,Tilt1,Tilt2
  固定翼混控 : Subsystem
  多旋翼混控 : Subsystem
  w1 : Outport
  w2 : Outport  Port=2
  w3 : Outport  Port=3
  tilt1 : Outport  Port=4
  tilt2 : Outport  Port=5
  dA1 : Outport  Port=6
  dA2 : Outport  Port=7
  wires:
  "FixedwingControlOutput "/1 -> 固定翼混控/2("FixedwingControlOutput ")
  固定翼混控/2(FixedwingCtrlSurface) -> Bus Selector/1
  "MultirotorControlOutput "/1 -> 多旋翼混控/2("MultirotorControlOutput ")
  固定翼混控/1(toMultirotorMixer) -> 多旋翼混控/4(toMultirotorMixer)
  Bus Selector/2 -> dA2/1  "<dA2>"
  Bus Selector/1 -> dA1/1  "<dA1>"
  多旋翼混控/1(MultirotorActuator) -> Bus Selector1/1
  Bus Selector1/1 -> w1/1  "<w1>"
  Bus Selector1/2 -> w2/1  "<w2>"
  Bus Selector1/3 -> w3/1  "<w3>"
  Bus Selector1/4 -> tilt1/1  "<Tilt1>"
  Bus Selector1/5 -> tilt2/1  "<Tilt2>"
  FlightMode/1 -> 多旋翼混控/3(FlightMode), 固定翼混控/1(FlightMode)
  States/1 -> 多旋翼混控/1(States)

== system Y3Tiltrotor_sim3_INDI/Y3 Tiltrotor Aircraft Model/States Bus ==
  Ve : Inport
  Xe : Inport  Port=2
  Euler : Inport  Port=3
  DCMbe : Inport  Port=4
  Vb : Inport  Port=5
  pqr : Inport  Port=6
  dw/dt : Inport  Port=7
  Abb : Inport  Port=8
  RotorParams : Inport  Port=9
  Airspeed : Inport  Port=10
  Direction Cosine Matrix to Quaternions : Dcm2Quat
  MATLAB Function1 : MATLAB Function  TreatAsAtomicUnit=on
  Reshape : Reshape  OutputDimensionality=Column vector (2-D)
  Reshape1 : Reshape  OutputDimensionality=Row vector (2-D)
  Selector : Selector  InputPortWidth=3  IndexOptions=Index vector (dialog)  Indices=[3 2 1]  OutputSizes=1
  Bus Element Out15 : Outport  PortName=States  Element=Ve
  Bus Element Out16 : Outport  PortName=States  Element=course
  Bus Element Out17 : Outport  PortName=States  Element=gndspeed
  Bus Element Out18 : Outport  PortName=States  Element=Xe
  Bus Element Out19 : Outport  PortName=States  Element=Euler
  Bus Element Out20 : Outport  PortName=States  Element=ypr
  Bus Element Out21 : Outport  PortName=States  Element=q
  Bus Element Out22 : Outport  PortName=States  Element=DCMbe
  Bus Element Out23 : Outport  PortName=States  Element=Vb
  Bus Element Out24 : Outport  PortName=States  Element=pqr
  Bus Element Out25 : Outport  PortName=States  Element=dw/dt
  Bus Element Out26 : Outport  PortName=States  Element=Abb
  Bus Element Out27 : Outport  PortName=States  Element=RotorParameters
  Bus Element Out28 : Outport  PortName=States  Element=Airspeed
  wires:
  DCMbe/1 -> Bus Element Out22/1, Direction Cosine Matrix to Quaternions/1
  Airspeed/1 -> Bus Element Out28/1
  Ve/1 -> Bus Element Out15/1, MATLAB Function1/1(vxyz)
  MATLAB Function1/1(course) -> Bus Element Out16/1  "course"
  MATLAB Function1/2(gndSpeed) -> Bus Element Out17/1  "gndspeed"
  Xe/1 -> Bus Element Out18/1
  Euler/1 -> Reshape/1
  Vb/1 -> Reshape1/1
  Direction Cosine Matrix to Quaternions/1 -> Bus Element Out21/1  "q"
  pqr/1 -> Bus Element Out24/1
  Abb/1 -> Bus Element Out26/1
  RotorParams/1 -> Bus Element Out27/1  "RotorParameters"
  Selector/1 -> Bus Element Out20/1
  Reshape/1 -> Bus Element Out19/1, Selector/1
  Reshape1/1 -> Bus Element Out23/1
  dw/dt/1 -> Bus Element Out25/1

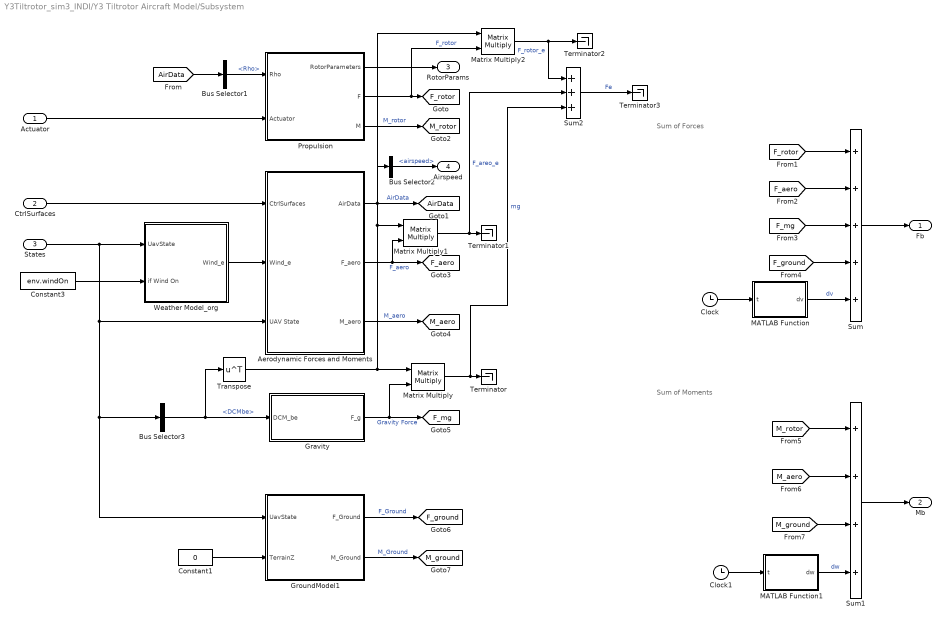
== system Y3Tiltrotor_sim3_INDI/Y3 Tiltrotor Aircraft Model/Subsystem ==
  note: Sum of Moments
  note: Sum of Forces
  Actuator : Inport
  CtrlSurfaces : Inport  Port=2
  States : Inport  Port=3
  Aerodynamic Forces and Moments : Subsystem
  Bus Selector1 : BusSelector  OutputSignals=Rho
  Bus Selector2 : BusSelector  OutputSignals=airspeed
  Bus Selector3 : BusSelector  OutputSignals=DCMbe
  Clock : Clock
  Clock1 : Clock
  Constant1 : Constant  Value=0
  Constant3 : Constant  Value=env.windOn
      settings: AttributesFormatString=%<Value>
  Gravity : Subsystem
  GroundModel1 : Subsystem
  MATLAB Function : MATLAB Function  TreatAsAtomicUnit=on
  MATLAB Function1 : MATLAB Function  TreatAsAtomicUnit=on
  Matrix Multiply : Product  Multiplication=Matrix(*)
  Matrix Multiply1 : Product  Multiplication=Matrix(*)
  Matrix Multiply2 : Product  Multiplication=Matrix(*)
  Propulsion : Subsystem
  Sum : Sum  Inputs=+++++
  Sum1 : Sum  Inputs=++++
  Sum2 : Sum  Inputs=+++
  Terminator{,1..3} (4 alike) : Terminator
  Transpose : Math  Operator=transpose
  Weather Model_org : Subsystem
  Fb : Outport
  Mb : Outport  Port=2
  RotorParams : Outport  Port=3
  Airspeed : Outport  Port=4
  tag scope: AirData=global, F_aero=global, F_ground=global, F_mg=global, F_rotor=global, M_aero=global, M_ground=global, M_rotor=global
  wires:
  Constant3/1 -> Weather Model_org/2(if Wind On)
  States/1 -> Aerodynamic Forces and Moments/3(UAV State), GroundModel1/1(UavState), Bus Selector3/1, Weather Model_org/1(UavState)
  Weather Model_org/1(Wind_e) -> Aerodynamic Forces and Moments/2(Wind_e)
  CtrlSurfaces/1 -> Aerodynamic Forces and Moments/1(CtrlSurfaces)
  Actuator/1 -> Propulsion/2(Actuator)
  Aerodynamic Forces and Moments/1(AirData) -> [AirData], Bus Selector2/1  "AirData"
  [AirData] -> Bus Selector1/1
  Bus Selector1/1 -> Propulsion/1(Rho)  "<Rho>"
  Propulsion/1(RotorParameters) -> RotorParams/1
  Propulsion/2(F) -> Matrix Multiply2/2, [F_rotor]  "F_rotor"
  Propulsion/3(M) -> [M_rotor]  "M_rotor"
  Aerodynamic Forces and Moments/2(F_aero) -> Matrix Multiply1/2, [F_aero]  "F_aero"
  Aerodynamic Forces and Moments/3(M_aero) -> [M_aero]  "M_aero"
  Gravity/1(F_g) -> Matrix Multiply/2, [F_mg]  "Gravity Force"
  Sum/1 -> Fb/1
  Bus Selector2/1 -> Airspeed/1  "<airspeed>"
  [F_rotor] -> Sum/1
  [F_mg] -> Sum/3
  [F_ground] -> Sum/4
  [M_ground] -> Sum1/3
  Bus Selector3/1 -> Transpose/1, Gravity/1(DCM_be)  "<DCMbe>"
  Constant1/1 -> GroundModel1/2("TerrainZ ")
  GroundModel1/2(M_Ground) -> [M_ground]  "M_Ground"
  GroundModel1/1(F_Ground) -> [F_ground]  "F_Ground"
  [M_rotor] -> Sum1/1
  Sum1/1 -> Mb/1
  [F_aero] -> Sum/2
  Transpose/1 -> Matrix Multiply1/1, Matrix Multiply2/1, Matrix Multiply/1
  Matrix Multiply/1 -> Sum2/3, Terminator/1  "mg"
  Matrix Multiply1/1 -> Sum2/2, Terminator1/1  "F_areo_e"
  Matrix Multiply2/1 -> Sum2/1, Terminator2/1  "F_rotor_e"
  Sum2/1 -> Terminator3/1  "Fe"
  [M_aero] -> Sum1/2
  MATLAB Function/1(dv) -> Sum/5  "dv"
  Clock/1 -> MATLAB Function/1(t)
  Clock1/1 -> MATLAB Function1/1(t)
  MATLAB Function1/1(dw) -> Sum1/4  "dw"

== system Y3Tiltrotor_sim3_INDI/Subsystem/固定翼模态/InputConditioning_altitude ==
  Ch1 : Inport
  Saturation1 : Saturate  UpperLimit=1  LowerLimit=-1
  deadzone3 : MATLAB Function  TreatAsAtomicUnit=on
  max_vz : Gain  Gain=control.maxClimbRate  OutDataTypeStr=Inherit: Inherit via back propagation
  vz_fw_d : Outport  VectorParamsAs1DForOutWhenUnconnected=off
  wires:
  max_vz/1 -> vz_fw_d/1
  deadzone3/1(y) -> Saturation1/1
  Ch1/1 -> deadzone3/1(u)
  Saturation1/1 -> max_vz/1

== system Y3Tiltrotor_sim3_INDI/Subsystem/固定翼模态/InputConditioning_speed ==
  Ch3 : Inport
  vx0 : Inport  Port=2
  Gain16 : Gain  Gain=control.FWmaxSpeed
  Saturation1 : Saturate  UpperLimit=1  LowerLimit=-1
  Sum1 : Sum  Inputs=|++
  deadzone3 : MATLAB Function  TreatAsAtomicUnit=on
  Speed_cmd : Outport  VectorParamsAs1DForOutWhenUnconnected=off
  wires:
  Ch3/1 -> deadzone3/1(u)
  deadzone3/1(y) -> Saturation1/1
  Gain16/1 -> Sum1/1
  Sum1/1 -> Speed_cmd/1
  vx0/1 -> Sum1/2
  Saturation1/1 -> Gain16/1

== system Y3Tiltrotor_sim3_INDI/Subsystem/固定翼模态/InputConditioning_stablelize ==
  Ch1 : Inport
  Ch2 : Inport  Port=2
  Ch3 : Inport  Port=3
  Ch4 : Inport  Port=4
  Constant : Constant
  Gain : Gain  Gain=0.5
  Gain13 : Gain  Gain=control.FWmaxPitch
  Gain14 : Gain  Gain=control.maxRoll
  Gain15 : Gain  Gain=control.maxYawRate
  Gain16 : Gain
  Saturation{1,7..9} (4 alike) : Saturate  UpperLimit=1  LowerLimit=-1
  Saturation10 : Saturate  UpperLimit=1  LowerLimit=0
  Sum : Sum  Inputs=|++
  deadzone0 : MATLAB Function  TreatAsAtomicUnit=on
  deadzone1 : MATLAB Function  TreatAsAtomicUnit=on
  deadzone2 : MATLAB Function  TreatAsAtomicUnit=on
  deadzone3 : MATLAB Function  TreatAsAtomicUnit=on
  Roll_cmd : Outport  VectorParamsAs1DForOutWhenUnconnected=off
  Pitch_cmd : Outport  Port=2  VectorParamsAs1DForOutWhenUnconnected=off
  YawRate_cmd : Outport  Port=3  VectorParamsAs1DForOutWhenUnconnected=off
  Thrust_cmd : Outport  Port=4  VectorParamsAs1DForOutWhenUnconnected=off
  wires:
  Saturation10/1 -> Gain16/1
  Saturation7/1 -> Gain15/1
  Saturation9/1 -> Gain14/1
  Saturation8/1 -> Gain13/1
  deadzone0/1(y) -> Saturation9/1
  deadzone1/1(y) -> Saturation8/1
  deadzone2/1(y) -> Saturation7/1
  Ch1/1 -> deadzone1/1(u)
  Ch3/1 -> deadzone3/1(u)
  Ch2/1 -> deadzone0/1(u)
  Ch4/1 -> deadzone2/1(u)
  deadzone3/1(y) -> Saturation1/1
  Sum/1 -> Gain/1
  Saturation1/1 -> Sum/1
  Gain/1 -> Saturation10/1
  Constant/1 -> Sum/2
  Gain13/1 -> Pitch_cmd/1
  Gain14/1 -> Roll_cmd/1
  Gain15/1 -> YawRate_cmd/1
  Gain16/1 -> Thrust_cmd/1
